simulink model "control_cartezian"  (R2024b)
settings: Solver=VariableStepAuto  StartTime=0.0  StopTime=10.0  RelTol=1e-3
settings Model: Creator=Edy  LastModifiedBy=Edy

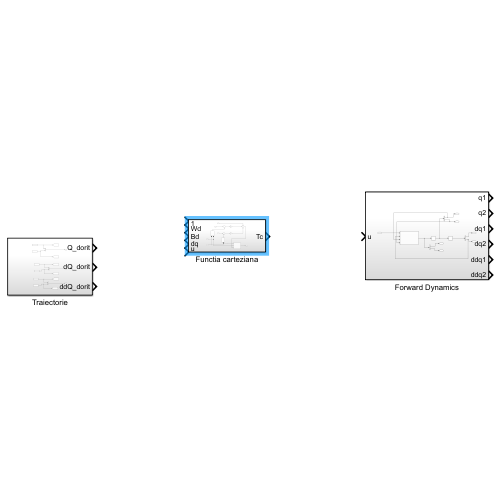
[thumbnail: Simulink's stored preview of the top-level diagram]
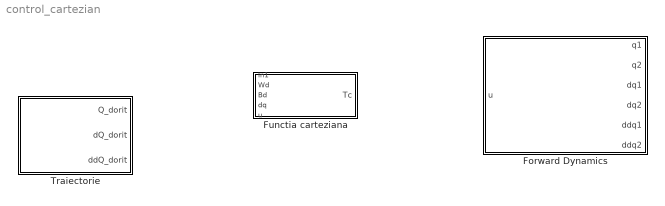
== system control_cartezian ==
  Forward Dynamics : Subsystem
  Functia carteziana : Subsystem
  Traiectorie : Subsystem

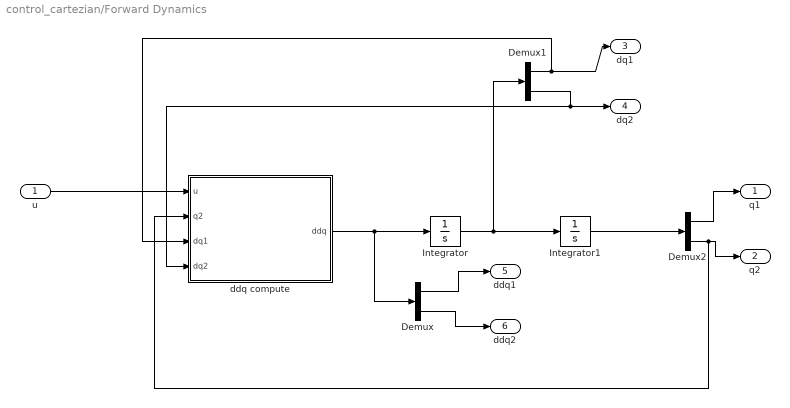
== system control_cartezian/Forward Dynamics ==
  u : Inport
  Demux : Demux  Outputs=2
  Demux1 : Demux  Outputs=2
  Demux2 : Demux  Outputs=2
  Integrator : Integrator
  Integrator1 : Integrator
  ddq compute : MATLAB Function  TreatAsAtomicUnit=on
  q1 : Outport
  q2 : Outport  Port=2
  dq1 : Outport  Port=3
  dq2 : Outport  Port=4
  ddq1 : Outport  Port=5
  ddq2 : Outport  Port=6
  wires:
  ddq compute/1(ddq) -> Demux/1, Integrator/1
  Integrator/1 -> Demux1/1, Integrator1/1
  Integrator1/1 -> Demux2/1
  Demux1/1 -> ddq compute/3(dq1), dq1/1
  Demux1/2 -> ddq compute/4(dq2), dq2/1
  u/1 -> ddq compute/1(u)
  Demux/1 -> ddq1/1
  Demux/2 -> ddq2/1
  Demux2/1 -> q1/1
  Demux2/2 -> ddq compute/2(q2), q2/1

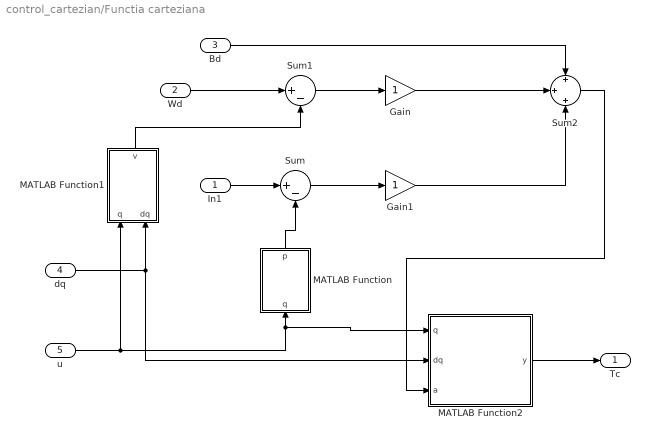
== system control_cartezian/Functia carteziana ==
  In1 : Inport
  Wd : Inport  Port=2
  Bd : Inport  Port=3
  dq : Inport  Port=4
  u : Inport  Port=5
  Gain : Gain
  Gain1 : Gain
  MATLAB Function : MATLAB Function  TreatAsAtomicUnit=on
  MATLAB Function1 : MATLAB Function  TreatAsAtomicUnit=on
  MATLAB Function2 : MATLAB Function  TreatAsAtomicUnit=on
  Sum : Sum  Inputs=|+-
  Sum1 : Sum  Inputs=|+-
  Sum2 : Sum  Inputs=+|+|+
  Tc : Outport
  wires:
  In1/1 -> Sum/1
  MATLAB Function/1(p) -> Sum/2
  u/1 -> MATLAB Function1/1(q), MATLAB Function2/1(q), MATLAB Function/1(q)
  Wd/1 -> Sum1/1
  MATLAB Function1/1(v) -> Sum1/2
  Sum1/1 -> Gain/1
  Bd/1 -> Sum2/1
  Gain/1 -> Sum2/2
  Sum/1 -> Gain1/1
  Gain1/1 -> Sum2/3
  MATLAB Function2/1(y) -> Tc/1
  dq/1 -> MATLAB Function1/2(dq), MATLAB Function2/2(dq)
  Sum2/1 -> MATLAB Function2/3(a)

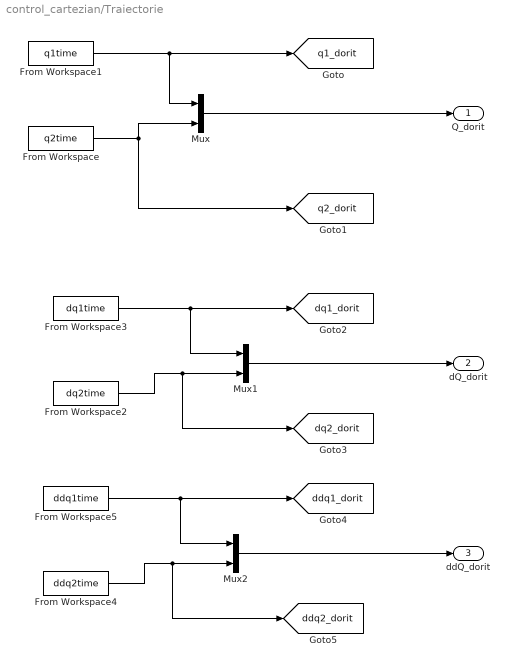
== system control_cartezian/Traiectorie ==
  From Workspace : FromWorkspace  VariableName=q2time
  From Workspace1 : FromWorkspace  VariableName=q1time
  From Workspace2 : FromWorkspace  VariableName=dq2time
  From Workspace3 : FromWorkspace  VariableName=dq1time
  From Workspace4 : FromWorkspace  VariableName=ddq2time
  From Workspace5 : FromWorkspace  VariableName=ddq1time
  Mux : Mux  Inputs=2
  Mux1 : Mux  Inputs=2
  Mux2 : Mux  Inputs=2
  Q_dorit : Outport
  dQ_dorit : Outport  Port=2
  ddQ_dorit : Outport  Port=3
  tag scope: ddq1_dorit=global, ddq2_dorit=global, dq1_dorit=global, dq2_dorit=global, q1_dorit=global, q2_dorit=global
  wires:
  Mux/1 -> Q_dorit/1
  From Workspace1/1 -> Mux/1, [q1_dorit]
  From Workspace/1 -> [q2_dorit], Mux/2
  From Workspace3/1 -> Mux1/1, [dq1_dorit]
  From Workspace2/1 -> [dq2_dorit], Mux1/2
  From Workspace4/1 -> [ddq2_dorit], Mux2/2
  From Workspace5/1 -> Mux2/1, [ddq1_dorit]
  Mux1/1 -> dQ_dorit/1
  Mux2/1 -> ddQ_dorit/1

== matlab function control_cartezian/Forward Dynamics/ddq compute ==
  data: u input; ddq output; q2 input; dq1 input; dq2 input
function ddq = forward_dynamics(u, q2, dq1, dq2)
    % =========================================================
    % 1. PARAMETRI STRUCTURA (R-T)
    % =========================================================
    m1 = 1;      
    m2 = 2;      
    l1 = 0.2;
    lc1 = 0.1;
    Izz1 = 3.68e-3;
    Izz2 = 7.366e-3;
    
    % =========================================================
    % 2. PARAMETRI MOTOR & TRANSMISIE
    % =========================================================
    % ATENTIE: J_t trebuie sa fie in kg*m^2! 
    % Daca in fisa e 72.8 g*cm^2, atunci e 72.8e-7 kg*m^2
    J_rotor = 72.8e-7; 
    
    i_r = 103;        % Raport reductor
    eta = 1/1.74;     % Randament (0.57)
    b_mot = 0.1;      % Frecare vascoasa la ax motor
    k_M = 27.3e-3;    % Constanta cuplu [Nm/A]
    R = 0.108;        % Rezistenta [Ohm]

    % Parametri Surub (Pt Cupla 2 - Translatie)
    pas_surub = 0.005; % [m]
    ht = pas_surub / (2*pi); % [m/rad] Constant de transmisie

    % =========================================================
    % 3. CALCUL FACTORI DE TRANSMISIE
    % =========================================================
    
    % Raportul de transformare a miscarii (Motor -> Brat)
    % Alpha 1: [rad_motor / rad_brat] = i_r
    % Alpha 2: [rad_motor / m_brat]   = i_r / ht
    alpha1 = i_r;
    alpha2 = i_r / ht;
    
    % Matricea de transformare (Diagonala)
    T_ratio = diag([alpha1, alpha2]); 

    % =========================================================
    % 4. DINAMICA BRATULUI (Mecanic)
    % =========================================================
    
    % Matricea de Inertie a Bratului M(q) - Specifica R-T
    M_brat = [m2*l1^2 + 2*m2*q2*l1 + m1*lc1^2 + m2*q2^2 + Izz1 + Izz2, 0; 
              0, m2];

    % Matricea Coriolis/Centrifugal C(q, dq)
    % Termeni specifici R-T (fara sin/cos la q2)
    Cn = [0, 0; 
         -m2*(l1 + q2), 0];
         
    B_coriolis_vec = [2*m2*(l1+q2); 
                      0];
                      
    % Fortele Nelineare Mecanice [Nm] si [N]
    N_mec = Cn*[dq1^2; dq2^2] + B_coriolis_vec*dq1*dq2;
    
    % Gravitatia (Zero in plan orizontal)
    G = [0; 0];

    % =========================================================
    % 5. ECUATIA TOTALA (Cuplaj Electric + Mecanic)
    % =========================================================
    % Ecuatia standard: M_total * ddq + N_total + B_total = Tau_generat
    
    % A. Inertia Totala (Brat + Rotor reflectat prin reductor)
    % Inertia rotorului se amplifica cu patratul raportului de transmisie!
    J_rotors_reflected = diag([J_rotor * alpha1^2 * eta, ...
                               J_rotor * alpha2^2 * eta]);
                           
    M_total = M_brat + J_rotors_reflected;
    
    % B. Forta generata de Tensiune (u)
    % Tau_mot = (k_M/R) * u ... apoi amplificat de reductor
    Gain_Force = (k_M / R) * eta;
    F_active = Gain_Force * T_ratio * u; 
    
    % C. Damping Total (Frecare Motor + Back-EMF) reflectat la brat
    % Back-EMF creeaza o franare proportionala cu viteza^2 (prin transmisie)
    Damp_coeff_motor = b_mot + (k_M^2 / R);
    
    % Matricea de damping reflectata
    B_total_mat = diag([Damp_coeff_motor * alpha1^2 * eta, ...
                        Damp_coeff_motor * alpha2^2 * eta]);
                    
    F_damping = B_total_mat * [dq1; dq2];
    
    % =========================================================
    % 6. CALCUL ACCELERATIE (ddq)
    % =========================================================
    
    % ddq = inv(M) * (Forte_Active - Nelinearitati - Damping - Gravitatie)
    ddq = M_total \ (F_active - N_mec - F_damping - G);

end

== matlab function control_cartezian/Functia carteziana/MATLAB Function ==
  data: q input; p output
function p = fcn(q)
    % Parametri geometrici
    l1 = 0.2; % Lungimea fixa a primei parti a bratului
    
    % Variabile
    q1 = q(1); % Unghiul de rotatie (radiani)
    q2 = q(2); % Extensia prismatica (metri)

    % Calculul pozitiei Carteziene (X, Y)
    % Raza totala r = l1 + q2
    
    % Pozitia pe axa X
    x = (l1 + q2) * cos(q1);
    
    % Pozitia pe axa Y
    y = (l1 + q2) * sin(q1);

    % Returnam vectorul pozitie
    p = [x; y];
end

== matlab function control_cartezian/Functia carteziana/MATLAB Function1 ==
  data: q input; v output; dq input
function v = fcn(q, dq)
    % Parametri geometrici
    l1 = 0.2; % Offset-ul fix al bratului
    
    % Extragere variabile de stare
    q1 = q(1); % Unghiul de rotatie (rad)
    q2 = q(2); % Extensia prismatica (m)
    
    % --- Matricea Jacobiana J(q) pentru R-T ---
    % Pozitia X = (l1 + q2) * cos(q1)
    % Pozitia Y = (l1 + q2) * sin(q1)
    
    % Derivatele partiale pentru Jacobian:
    % J11 = dX/dq1 = -(l1+q2)*sin(q1)
    % J12 = dX/dq2 = cos(q1)
    % J21 = dY/dq1 = (l1+q2)*cos(q1)
    % J22 = dY/dq2 = sin(q1)
    
    J = [ -(l1 + q2)*sin(q1),   cos(q1);
           (l1 + q2)*cos(q1),   sin(q1) ];
       
    % Calculul vitezei carteziene (v_x, v_y)
    % v = J * dq
    v = J * [dq(1); dq(2)];
end

== matlab function control_cartezian/Functia carteziana/MATLAB Function2 ==
  data: q input; y output; dq input; a input
function y = fcn(q, dq, a)
y = u;
